simulink model "Setpointprovider"  (R2024b)
settings: Solver=FixedStepAuto  StartTime=0.0  StopTime=50.0  FixedStep=0.02  MaxStep=1e-3  RelTol=1e-3  EnableMultiTasking=on
model workspace (MAT data in the model file):
  Kd = 10
  Kr = 0
  L = 0.5
  a = 12.5
  b = 16
  c = 14
  g = 9.81
  lp = 0.62
  mCart = 2
  mPend = 0.0812
  rp = 5
  theta0 = 0
settings Model: Creator=The MathWorks, Inc.  LastModifiedBy=eduar
settings SolverCC: AlgebraicLoopSolver=TrustRegion
settings DataIOCC: SaveFormat=Array  SaveOutput=off  SaveTime=off  ReturnWorkspaceOutputs=off  OutputTimes=0:1/30:50
settings OptimizationCC: ReuseModelBlockBuffer=off  LifeSpan=inf
settings DebuggingCC: UnderspecifiedInitializationDetection=Classic  MergeDetectMultiDrivingBlocksExec=none  SolverPrmCheckMsg=warning  UnconnectedInputMsg=warning  UnconnectedOutputMsg=warning  UnconnectedLineMsg=warning  StateNameClashWarn=warning  SFUnexpectedBacktrackingDiag=warning  SFNoUnconditionalDefaultTransitionDiag=warning  SFExecutionAtInitializationDiag=none  ArithmeticOperatorsInVariantConditions=warning
settings HardwareCC: ProdBitPerPointer=32  ProdBitPerSizeT=32  ProdBitPerPtrDiffT=32  ProdLargestAtomicFloat=None  ProdIntDivRoundTo=Undefined  ProdEndianess=Unspecified  ProdWordSize=32  ProdHWDeviceType=32-bit Generic
settings ModelReferenceCC: EnableRefExpFcnMdlSchedulingChecks=on  PropagateSignalLabelsOutOfModel=off
settings SFSimCC: SimUseLocalCustomCode=off  CustomCodeUndefinedFunction=UseInterfaceOnly
settings RTWCC: RTWUseLocalCustomCode=off  GPUComputeCapability=3.5
settings CodeAppCC: StateflowObjectComments=on
settings GRTTargetCC: TargetLangStandard=C89/C90 (ANSI)
settings ConfigComp: CovMetricSettings=dw  CovSaveCumulativeToWorkspaceVar=on  CovSaveSingleToWorkspaceVar=on  CovExternalEMLEnable=off  CovSFcnEnable=off
settings SimscapeCC: SimscapeNormalizeSystem=off
settings ConfigurationSet: Description=SimMechanics 2G
settings ExplorerConfigSet: InternalSimMechanicsExplorerSettings="<ExplorerConfiguration><canonicalview>default</canonicalview><TilePanel><TileInfo><Tiles Columns=\"1\" Count=\"1\" Rows=\"1\"><Column Left=\"2\" Weight=\"1\"/><Column Left=\"591\"/><Row Top=\"2\" Weight=\"1\"/><Row Top=\"389\"/><Tile Height=\"1\" Width=\"1\" X=\"0\" Y=\"0\"/></Tiles></TileInfo><SceneInfo><SceneViewer><BGColor><R>0.60000002384185791</R><G>0.60000002384185791</G><B>0.60000002384185791</B></BGColor><Camera><Position><X>0.64243946887929204</X><Y>-49.663614699976236</Y><Z>0.22319801622928798</Z></Position><Center><X>0.64243946887929204</X><Y>0</Y><Z>0.22319801622928798</Z></Center><Up><X>0</X><Y>-0</Y><Z>1</Z></Up><Left>-0.88124258449330872</Left><Right>0.88124258449330872</Right><Bottom>-0.30475961919215644</Bottom><Top>0.30475961919215644</Top></Camera></SceneViewer></SceneInfo></TilePanel></ExplorerConfiguration>"

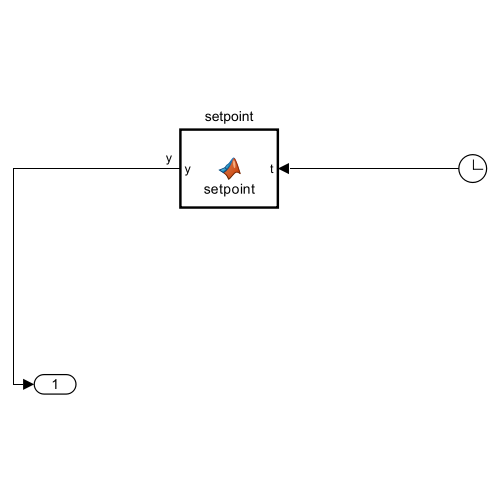
[thumbnail: Simulink's stored preview of the top-level diagram]
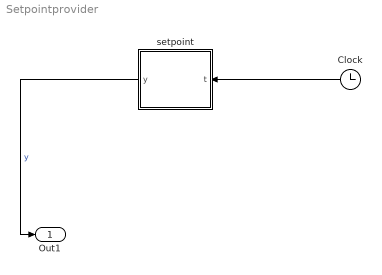
== system Setpointprovider ==
  Clock : Clock
  setpoint : MATLAB Function  TreatAsAtomicUnit=on
  Out1 : Outport  OutDataTypeStr=double  PortDimensions=1  SampleTime=0  VectorParamsAs1DForOutWhenUnconnected=off
  wires:
  Clock/1 -> setpoint/1(t)
  setpoint/1(y) -> Out1/1  "y"

== matlab function Setpointprovider/setpoint ==
  data: t input; y output
function y = setpoint(t)

sp = [1 2 1 2 3 2 3 4 3 4 5 4];

pos = floor(t/5)+1;

y = sp(pos);
